simulink model "MOBATSim"  (R2020b)
settings: Solver=FixedStepAuto  StartTime=0.0  StopTime=Sim_t  FixedStep=0.01  MinStep=0.01  RelTol=1e-2
values from neighbouring files (symbols this model uses):
  Vehicles = evalin('base','Vehicles')    [I2V.m]    (also in VehicleSensors.m)
undefined symbols (not defined in the file or in its folder): Sim_Ts
libraries: simulink x50, robotalgslib x10, drivingvehiclecontroller x10, mpcadaslib x10, pid_lib x10
(part 2 of 7)

== system MOBATSim/Vehicle Model 9 ==
  note: Perception
  note: Decision-Making
  note: Control
  Behavioural Planner : MATLABSystem  System=VehicleDrivingMode  Vehicle_id=Vehicle_id  SimulateUsing=Interpreted execution
      mask Type: VehicleDrivingMode
      mask Display:
      | image('MOBATSIM-Icon-Set_7- Behavioural Planner.png');
      | port_label('input',1,'vehicleDetected');
      | port_label('output',1,'SpeedReference');
      | port_label('output',2,'DistanceReference');
      | port_label('output',3,'LeadSpeed');
      | port_label('output',4,'DrivingMode');
      | port_label('output',5,'Dist2Stop');
      | port_label('output',6,'laneChange');
  Longitudinal and Lateral Controllers : Subsystem
  Path Planner : Subsystem  Variant=on  VariantControlMode=label  LabelModeActiveChoice=Astar  mask{PathPlanningAlgorithm=Astar}
      mask prompts: PathPlanningAlgorithm "Path Planning Algorithm"
      mask TypeOptions PathPlanningAlgorithm: Astar | ShortestPathFinder
      mask Callback PathPlanningAlgorithm: set_param(gcb,'OverrideUsingVariant',get_param(gcb,'PathPlanningAlgorithm'));
      mask Display: image("MOBATSIM-Icon-Set_8- Navigation.png");
  Transform to MOBATSim Coordinates : Subsystem
  Vehicle Model : Subsystem  mask{Vehicle_id=Vehicle_id}
      mask prompts: Vehicle_id "Vehicle ID"
      mask Display: image('MOBATSIM-Icon-Set_13- VehicleModel.png'); % Use "Edit Image" on toolstrip to change.
  Vehicle Sensors : MATLABSystem  System=VehicleSensors  Vehicle_id=Vehicle_id  Tsample=Sim_Ts  OffsetTime=0  SimulateUsing=Interpreted execution
      mask Type: VehicleSensors
      mask Display:
      | image('MOBATSIM-Icon-Set_4- Sensor.png');
      | port_label('output',1,'V2VcommIDs');
      | port_label('output',2,'vehicleDetected');
  Vehicle Status Check and Acceleration to Speed : Subsystem
  Vehicle V2I Output : MATLABSystem  System=VehicleV2I_Out  Vehicle_id=Vehicle_id  SimulateUsing=Interpreted execution
      mask Type: VehicleV2I_Out
      mask Display:
      | image('MOBATSIM-Icon-Set_6- V2l.png');
      | port_label('input',1,'waypointReached');
      | port_label('output',1,'V2Idata');
  Position : Outport  VectorParamsAs1DForOutWhenUnconnected=off
  Orientation : Outport  Port=2  VectorParamsAs1DForOutWhenUnconnected=off
  Speed : Outport  Port=3  VectorParamsAs1DForOutWhenUnconnected=off
  V_Network_Out : Outport  Port=4  VectorParamsAs1DForOutWhenUnconnected=off
  wires:
  Vehicle V2I Output/1 -> V_Network_Out/1
  Vehicle Sensors/2 -> Behavioural Planner/1
  Behavioural Planner/1 -> Longitudinal and Lateral Controllers/1(Speed Reference)
  Behavioural Planner/2 -> Longitudinal and Lateral Controllers/2(Inter Vehicular Distance)
  Behavioural Planner/3 -> Longitudinal and Lateral Controllers/3(Lead Speed)
  Behavioural Planner/4 -> Longitudinal and Lateral Controllers/4(drivingMode)
  Behavioural Planner/5 -> Longitudinal and Lateral Controllers/5(Dist2Stop)
  Transform to MOBATSim Coordinates/1(Position) -> Position/1
  Transform to MOBATSim Coordinates/2(Orientation) -> Orientation/1
  Vehicle Model/2(Speed) -> Longitudinal and Lateral Controllers/8(Actual Speed), Speed/1
  Vehicle Model/1(Pose) -> Longitudinal and Lateral Controllers/7(Actual Pose), Transform to MOBATSim Coordinates/1(Pose)
  Longitudinal and Lateral Controllers/1(Longitudinal Acceleration Cmd) -> Vehicle Status Check and Acceleration to Speed/1(Reference Acceleration)
  Longitudinal and Lateral Controllers/2(Reference Steering Angle) -> Vehicle Status Check and Acceleration to Speed/2(Reference Steering Angle)
  Vehicle Status Check and Acceleration to Speed/2(Steering Angle Cmd) -> Vehicle Model/2(Steering Angle)
  Behavioural Planner/6 -> Longitudinal and Lateral Controllers/6(laneChange)
  Vehicle Sensors/1 -> Path Planner/1(CommunicationIDs)
  Path Planner/1(waypointReached) -> Vehicle V2I Output/1
  Vehicle Status Check and Acceleration to Speed/1(Speed Cmd) -> Vehicle Model/1(Longitudinal Speed)

== system MOBATSim/Vehicle Model 1/Longitudinal and Lateral Controllers ==
  Speed Reference : Inport
  Inter Vehicular Distance : Inport  Port=2
  Lead Speed : Inport  Port=3
  drivingMode : Inport  Port=4
  Dist2Stop : Inport  Port=5
  laneChange : Inport  Port=6
  Actual Pose : Inport  Port=7
  Actual Speed : Inport  Port=8
  Lateral Motion Control : Subsystem  Variant=on  VariantControlMode=label  LabelModeActiveChoice=STANLEY  mask{modeLateral=STANLEY}
      mask prompts: modeLateral "Lateral Control Mode:"
      mask TypeOptions modeLateral: PURE_PURSUIT | STANLEY
      mask Callback modeLateral: set_param(gcb,'OverrideUsingVariant',get_param(gcb,'modeLateral'));
  Longitudinal Speed Control : Subsystem
  Longitudinal Acceleration Cmd : Outport
  Reference Steering Angle : Outport  Port=2
  wires:
  laneChange/1 -> Lateral Motion Control/3(changeLane)
  Lateral Motion Control/1(SteerCmd) -> Reference Steering Angle/1
  Actual Speed/1 -> Lateral Motion Control/1(speed), Longitudinal Speed Control/6(Actual Speed)
  drivingMode/1 -> Longitudinal Speed Control/4(Driving Mode)
  Longitudinal Speed Control/1(Longitduinal Acceleration Command) -> Longitudinal Acceleration Cmd/1
  Dist2Stop/1 -> Longitudinal Speed Control/5(Dist2Stop)
  Inter Vehicular Distance/1 -> Longitudinal Speed Control/2(Inter Vehicular Distance)
  Lead Speed/1 -> Longitudinal Speed Control/3(Lead Speed)
  Speed Reference/1 -> Longitudinal Speed Control/1(Speed Reference)
  Actual Pose/1 -> Lateral Motion Control/2(pose)

== system MOBATSim/Vehicle Model 1/Path Planner ==
  note: 1) Add Subsystem or Model blocks as valid variant choices.
      | 2) You cannot connect blocks at this level. At simulation, connectivity is automatically
      | determined, based on the active variant and port name matching.
  CommunicationIDs : Inport
  Astar : Subsystem  VariantControl=Astar
  ShortestPathFinder : Subsystem  VariantControl=ShortestPathFinder
  waypointReached : Outport

== system MOBATSim/Vehicle Model 1/Transform to MOBATSim Coordinates ==
  Pose : Inport
  Constant : Constant  Value=0
  Constant1 : Constant
  Constant2 : Constant  Value=0
  Constant3 : Constant  Value=0
  Constant4 : Constant  Value=pi/2
  Gain : Gain  Gain=-1
  Matrix Concatenate : Concatenate  NumInputs=4  ConcatenateDimension=2
  Matrix Concatenate1 : Concatenate  NumInputs=3  ConcatenateDimension=2
  Selector1 : Selector  InputPortWidth=3  IndexOptions=Index vector (dialog)  Indices=[3]  OutputSizes=1
  Selector3 : Selector  InputPortWidth=3  IndexOptions=Index vector (dialog)  Indices=[1]  OutputSizes=1
  Selector4 : Selector  InputPortWidth=3  IndexOptions=Index vector (dialog)  Indices=[2]  OutputSizes=1
  Sum : Sum  Inputs=|++
  Position : Outport
  Orientation : Outport  Port=2
  wires:
  Sum/1 -> Matrix Concatenate/4
  Constant2/1 -> Matrix Concatenate/1
  Constant3/1 -> Matrix Concatenate1/2
  Gain/1 -> Matrix Concatenate1/3
  Constant4/1 -> Sum/2
  Constant1/1 -> Matrix Concatenate/2
  Selector1/1 -> Sum/1
  Constant/1 -> Matrix Concatenate/3
  Matrix Concatenate/1 -> Orientation/1
  Matrix Concatenate1/1 -> Position/1
  Selector4/1 -> Gain/1
  Selector3/1 -> Matrix Concatenate1/1
  Pose/1 -> Selector1/1, Selector4/1, Selector3/1

== system MOBATSim/Vehicle Model 1/Vehicle Model ==
  Longitudinal Speed : Inport
  Steering Angle : Inport  Port=2
  Delay : Delay  DelayLength=1  SampleTime=Sim_Ts
  Kinematic Bicycle Model : Subsystem
  Selector3 : Selector  InputPortWidth=3  IndexOptions=Index vector (dialog)  Indices=[1]  OutputSizes=1
  Selector4 : Selector  InputPortWidth=3  IndexOptions=Index vector (dialog)  Indices=[2]  OutputSizes=1
  Sqrt : Sqrt  SaturateOnIntegerOverflow=on
  Square : Math  Operator=square  SaturateOnIntegerOverflow=on
  Square1 : Math  Operator=square  SaturateOnIntegerOverflow=on
  Sum1 : Sum  Inputs=|++
  Zero-Order Hold1 : ZeroOrderHold  SampleTime=Sim_Ts
  Zero-Order Hold2 : ZeroOrderHold  SampleTime=Sim_Ts
  Pose : Outport
  Speed : Outport  Port=2
  wires:
  Delay/1 -> Speed/1
  Kinematic Bicycle Model/1(state) -> Zero-Order Hold1/1
  Selector4/1 -> Square1/1
  Longitudinal Speed/1 -> Kinematic Bicycle Model/1(v)
  Steering Angle/1 -> Kinematic Bicycle Model/2(Steering Angle)
  Sum1/1 -> Sqrt/1
  Sqrt/1 -> Delay/1
  Square/1 -> Sum1/1
  Square1/1 -> Sum1/2
  Selector3/1 -> Square/1
  Kinematic Bicycle Model/2(stateDot) -> Zero-Order Hold2/1
  Zero-Order Hold1/1 -> Pose/1
  Zero-Order Hold2/1 -> Selector4/1, Selector3/1

== system MOBATSim/Vehicle Model 1/Vehicle Status Check and Acceleration to Speed ==
  note: Longitudinal
  Reference Acceleration : Inport
  Reference Steering Angle : Inport  Port=2
  Acceleration to Speed : Integrator  LimitOutput=on  LowerSaturationLimit=0
  MATLAB System : MATLABSystem  System=VehicleStopStatusCheck  Vehicle_id=Vehicle_id  SimulateUsing=Interpreted execution
      mask Type: VehicleStopStatusCheck
      mask Display:
      | disp('VehicleStopStatusCheck');
      | port_label('input',1,'Acc');
      | port_label('input',2,'Steering');
      | port_label('output',1,'Acc');
      | port_label('output',2,'Stop');
      | port_label('output',3,'Steering');
  Product : Product
  Signal Specification : SignalSpecification  Dimensions=1
  Stop Check : simulink/Logic and Bit Operations/Compare To Constant  relop=~=  const=1  OutDataTypeStr=uint8
  Zero-Order Hold : ZeroOrderHold  SampleTime=Sim_Ts
  Speed Cmd : Outport
  Steering Angle Cmd : Outport  Port=2
  wires:
  Acceleration to Speed/1 -> Signal Specification/1
  Stop Check/1 -> Product/2
  MATLAB System/3 -> Steering Angle Cmd/1
  Signal Specification/1 -> Zero-Order Hold/1
  Reference Acceleration/1 -> MATLAB System/1
  Zero-Order Hold/1 -> Product/1
  Product/1 -> Speed Cmd/1
  MATLAB System/1 -> Acceleration to Speed/1
  Reference Steering Angle/1 -> MATLAB System/2
  MATLAB System/2 -> Stop Check/1

== system MOBATSim/Vehicle Model 10/Longitudinal and Lateral Controllers ==
  Speed Reference : Inport
  Inter Vehicular Distance : Inport  Port=2
  Lead Speed : Inport  Port=3
  drivingMode : Inport  Port=4
  Dist2Stop : Inport  Port=5
  laneChange : Inport  Port=6
  Actual Pose : Inport  Port=7
  Actual Speed : Inport  Port=8
  Lateral Motion Control : Subsystem  Variant=on  VariantControlMode=label  LabelModeActiveChoice=STANLEY  mask{modeLateral=STANLEY}
      mask prompts: modeLateral "Lateral Control Mode:"
      mask TypeOptions modeLateral: PURE_PURSUIT | STANLEY
      mask Callback modeLateral: set_param(gcb,'OverrideUsingVariant',get_param(gcb,'modeLateral'));
  Longitudinal Speed Control : Subsystem
  Longitudinal Acceleration Cmd : Outport
  Reference Steering Angle : Outport  Port=2
  wires:
  laneChange/1 -> Lateral Motion Control/3(changeLane)
  Lateral Motion Control/1(SteerCmd) -> Reference Steering Angle/1
  Actual Speed/1 -> Lateral Motion Control/1(speed), Longitudinal Speed Control/6(Actual Speed)
  drivingMode/1 -> Longitudinal Speed Control/4(Driving Mode)
  Longitudinal Speed Control/1(Longitduinal Acceleration Command) -> Longitudinal Acceleration Cmd/1
  Dist2Stop/1 -> Longitudinal Speed Control/5(Dist2Stop)
  Inter Vehicular Distance/1 -> Longitudinal Speed Control/2(Inter Vehicular Distance)
  Lead Speed/1 -> Longitudinal Speed Control/3(Lead Speed)
  Speed Reference/1 -> Longitudinal Speed Control/1(Speed Reference)
  Actual Pose/1 -> Lateral Motion Control/2(pose)

== system MOBATSim/Vehicle Model 10/Path Planner ==
  note: 1) Add Subsystem or Model blocks as valid variant choices.
      | 2) You cannot connect blocks at this level. At simulation, connectivity is automatically
      | determined, based on the active variant and port name matching.
  CommunicationIDs : Inport
  Astar : Subsystem  VariantControl=Astar
  ShortestPathFinder : Subsystem  VariantControl=ShortestPathFinder
  waypointReached : Outport

== system MOBATSim/Vehicle Model 10/Transform to MOBATSim Coordinates ==
  Pose : Inport
  Constant : Constant  Value=0
  Constant1 : Constant
  Constant2 : Constant  Value=0
  Constant3 : Constant  Value=0
  Constant4 : Constant  Value=pi/2
  Gain : Gain  Gain=-1
  Matrix Concatenate : Concatenate  NumInputs=4  ConcatenateDimension=2
  Matrix Concatenate1 : Concatenate  NumInputs=3  ConcatenateDimension=2
  Selector1 : Selector  InputPortWidth=3  IndexOptions=Index vector (dialog)  Indices=[3]  OutputSizes=1
  Selector3 : Selector  InputPortWidth=3  IndexOptions=Index vector (dialog)  Indices=[1]  OutputSizes=1
  Selector4 : Selector  InputPortWidth=3  IndexOptions=Index vector (dialog)  Indices=[2]  OutputSizes=1
  Sum : Sum  Inputs=|++
  Position : Outport
  Orientation : Outport  Port=2
  wires:
  Sum/1 -> Matrix Concatenate/4
  Constant2/1 -> Matrix Concatenate/1
  Constant3/1 -> Matrix Concatenate1/2
  Gain/1 -> Matrix Concatenate1/3
  Constant4/1 -> Sum/2
  Constant1/1 -> Matrix Concatenate/2
  Selector1/1 -> Sum/1
  Constant/1 -> Matrix Concatenate/3
  Matrix Concatenate/1 -> Orientation/1
  Matrix Concatenate1/1 -> Position/1
  Selector4/1 -> Gain/1
  Selector3/1 -> Matrix Concatenate1/1
  Pose/1 -> Selector1/1, Selector4/1, Selector3/1

== system MOBATSim/Vehicle Model 10/Vehicle Model ==
  Longitudinal Speed : Inport
  Steering Angle : Inport  Port=2
  Delay : Delay  DelayLength=1  SampleTime=Sim_Ts
  Kinematic Bicycle Model : Subsystem
  Selector3 : Selector  InputPortWidth=3  IndexOptions=Index vector (dialog)  Indices=[1]  OutputSizes=1
  Selector4 : Selector  InputPortWidth=3  IndexOptions=Index vector (dialog)  Indices=[2]  OutputSizes=1
  Sqrt : Sqrt  SaturateOnIntegerOverflow=on
  Square : Math  Operator=square  SaturateOnIntegerOverflow=on
  Square1 : Math  Operator=square  SaturateOnIntegerOverflow=on
  Sum1 : Sum  Inputs=|++
  Zero-Order Hold1 : ZeroOrderHold  SampleTime=Sim_Ts
  Zero-Order Hold2 : ZeroOrderHold  SampleTime=Sim_Ts
  Pose : Outport
  Speed : Outport  Port=2
  wires:
  Delay/1 -> Speed/1
  Kinematic Bicycle Model/1(state) -> Zero-Order Hold1/1
  Selector4/1 -> Square1/1
  Longitudinal Speed/1 -> Kinematic Bicycle Model/1(v)
  Steering Angle/1 -> Kinematic Bicycle Model/2(Steering Angle)
  Sum1/1 -> Sqrt/1
  Sqrt/1 -> Delay/1
  Square/1 -> Sum1/1
  Square1/1 -> Sum1/2
  Selector3/1 -> Square/1
  Kinematic Bicycle Model/2(stateDot) -> Zero-Order Hold2/1
  Zero-Order Hold1/1 -> Pose/1
  Zero-Order Hold2/1 -> Selector4/1, Selector3/1

== system MOBATSim/Vehicle Model 10/Vehicle Status Check and Acceleration to Speed ==
  note: Longitudinal
  Reference Acceleration : Inport
  Reference Steering Angle : Inport  Port=2
  Acceleration to Speed : Integrator  LimitOutput=on  LowerSaturationLimit=0
  MATLAB System : MATLABSystem  System=VehicleStopStatusCheck  Vehicle_id=Vehicle_id  SimulateUsing=Interpreted execution
      mask Type: VehicleStopStatusCheck
      mask Display:
      | disp('VehicleStopStatusCheck');
      | port_label('input',1,'Acc');
      | port_label('input',2,'Steering');
      | port_label('output',1,'Acc');
      | port_label('output',2,'Stop');
      | port_label('output',3,'Steering');
  Product : Product
  Signal Specification : SignalSpecification  Dimensions=1
  Stop Check : simulink/Logic and Bit Operations/Compare To Constant  relop=~=  const=1  OutDataTypeStr=uint8
  Zero-Order Hold : ZeroOrderHold  SampleTime=Sim_Ts
  Speed Cmd : Outport
  Steering Angle Cmd : Outport  Port=2
  wires:
  Acceleration to Speed/1 -> Signal Specification/1
  Stop Check/1 -> Product/2
  MATLAB System/3 -> Steering Angle Cmd/1
  Signal Specification/1 -> Zero-Order Hold/1
  Reference Acceleration/1 -> MATLAB System/1
  Zero-Order Hold/1 -> Product/1
  Product/1 -> Speed Cmd/1
  MATLAB System/1 -> Acceleration to Speed/1
  Reference Steering Angle/1 -> MATLAB System/2
  MATLAB System/2 -> Stop Check/1

== system MOBATSim/Vehicle Model 2/Longitudinal and Lateral Controllers ==
  Speed Reference : Inport
  Inter Vehicular Distance : Inport  Port=2
  Lead Speed : Inport  Port=3
  Driving Mode : Inport  Port=4
  Dist2Stop : Inport  Port=5
  laneChange : Inport  Port=6
  Actual Pose : Inport  Port=7
  Actual Speed : Inport  Port=8
  Lateral Motion Control : Subsystem  Variant=on  VariantControlMode=label  LabelModeActiveChoice=STANLEY  mask{modeLateral=STANLEY}
      mask prompts: modeLateral "Lateral Control Mode:"
      mask TypeOptions modeLateral: PURE_PURSUIT | STANLEY
      mask Callback modeLateral: set_param(gcb,'OverrideUsingVariant',get_param(gcb,'modeLateral'));
  Longitudinal Speed Control : Subsystem
  Longitudinal Acceleration Cmd : Outport
  Reference Steering Angle : Outport  Port=2
  wires:
  Driving Mode/1 -> Longitudinal Speed Control/4(Driving Mode)
  Inter Vehicular Distance/1 -> Longitudinal Speed Control/2(Inter Vehicular Distance)
  Speed Reference/1 -> Longitudinal Speed Control/1(Speed Reference)
  Lead Speed/1 -> Longitudinal Speed Control/3(Lead Speed)
  Dist2Stop/1 -> Longitudinal Speed Control/5(Dist2Stop)
  Actual Speed/1 -> Lateral Motion Control/1(speed), Longitudinal Speed Control/6(Actual Speed)
  Longitudinal Speed Control/1(Longitduinal Acceleration Command) -> Longitudinal Acceleration Cmd/1
  laneChange/1 -> Lateral Motion Control/3(changeLane)
  Actual Pose/1 -> Lateral Motion Control/2(pose)
  Lateral Motion Control/1(SteerCmd) -> Reference Steering Angle/1

== system MOBATSim/Vehicle Model 2/Path Planner ==
  note: 1) Add Subsystem or Model blocks as valid variant choices.
      | 2) You cannot connect blocks at this level. At simulation, connectivity is automatically
      | determined, based on the active variant and port name matching.
  CommunicationIDs : Inport
  Astar : Subsystem  VariantControl=Astar
  ShortestPathFinder : Subsystem  VariantControl=ShortestPathFinder
  waypointReached : Outport

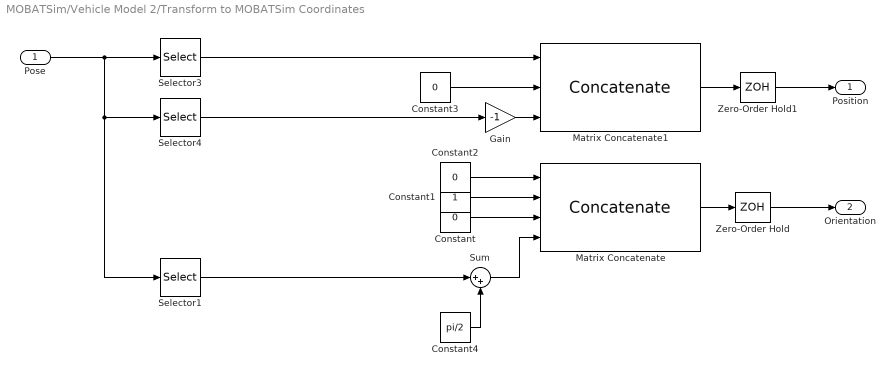
== system MOBATSim/Vehicle Model 2/Transform to MOBATSim Coordinates ==
  Pose : Inport
  Constant : Constant  Value=0
  Constant1 : Constant
  Constant2 : Constant  Value=0
  Constant3 : Constant  Value=0
  Constant4 : Constant  Value=pi/2
  Gain : Gain  Gain=-1
  Matrix Concatenate : Concatenate  NumInputs=4  ConcatenateDimension=2
  Matrix Concatenate1 : Concatenate  NumInputs=3  ConcatenateDimension=2
  Selector1 : Selector  InputPortWidth=3  IndexOptions=Index vector (dialog)  Indices=[3]  OutputSizes=1
  Selector3 : Selector  InputPortWidth=3  IndexOptions=Index vector (dialog)  Indices=[1]  OutputSizes=1
  Selector4 : Selector  InputPortWidth=3  IndexOptions=Index vector (dialog)  Indices=[2]  OutputSizes=1
  Sum : Sum  Inputs=|++
  Zero-Order Hold : ZeroOrderHold  SampleTime=Sim_Ts
  Zero-Order Hold1 : ZeroOrderHold  SampleTime=Sim_Ts
  Position : Outport
  Orientation : Outport  Port=2
  wires:
  Sum/1 -> Matrix Concatenate/4
  Constant2/1 -> Matrix Concatenate/1
  Matrix Concatenate/1 -> Zero-Order Hold/1
  Constant3/1 -> Matrix Concatenate1/2
  Gain/1 -> Matrix Concatenate1/3
  Constant4/1 -> Sum/2
  Constant1/1 -> Matrix Concatenate/2
  Matrix Concatenate1/1 -> Zero-Order Hold1/1
  Selector1/1 -> Sum/1
  Constant/1 -> Matrix Concatenate/3
  Zero-Order Hold/1 -> Orientation/1
  Zero-Order Hold1/1 -> Position/1
  Selector4/1 -> Gain/1
  Selector3/1 -> Matrix Concatenate1/1
  Pose/1 -> Selector1/1, Selector4/1, Selector3/1

== system MOBATSim/Vehicle Model 2/Vehicle Model ==
  Longitudinal Speed : Inport
  Steering Angle : Inport  Port=2
  Delay : Delay  DelayLength=1  SampleTime=Sim_Ts
  Kinematic Bicycle Model : Subsystem
  Selector3 : Selector  InputPortWidth=3  IndexOptions=Index vector (dialog)  Indices=[1]  OutputSizes=1
  Selector4 : Selector  InputPortWidth=3  IndexOptions=Index vector (dialog)  Indices=[2]  OutputSizes=1
  Sqrt : Sqrt  SaturateOnIntegerOverflow=on
  Square : Math  Operator=square  SaturateOnIntegerOverflow=on
  Square1 : Math  Operator=square  SaturateOnIntegerOverflow=on
  Sum1 : Sum  Inputs=|++
  Zero-Order Hold1 : ZeroOrderHold  SampleTime=Sim_Ts
  Zero-Order Hold2 : ZeroOrderHold  SampleTime=Sim_Ts
  Pose : Outport
  Speed : Outport  Port=2
  wires:
  Delay/1 -> Speed/1
  Kinematic Bicycle Model/1(state) -> Zero-Order Hold1/1
  Selector4/1 -> Square1/1
  Longitudinal Speed/1 -> Kinematic Bicycle Model/1(v)
  Steering Angle/1 -> Kinematic Bicycle Model/2(Steering Angle)
  Sum1/1 -> Sqrt/1
  Sqrt/1 -> Delay/1
  Square/1 -> Sum1/1
  Square1/1 -> Sum1/2
  Selector3/1 -> Square/1
  Kinematic Bicycle Model/2(stateDot) -> Zero-Order Hold2/1
  Zero-Order Hold1/1 -> Pose/1
  Zero-Order Hold2/1 -> Selector4/1, Selector3/1

== system MOBATSim/Vehicle Model 2/Vehicle Status Check and Acceleration to Speed ==
  note: Longitudinal
  Reference Acceleration : Inport
  Reference Steering Angle : Inport  Port=2
  Acceleration to Speed : Integrator  LimitOutput=on  UpperSaturationLimit=Vehicles(Vehicle_id).dynamics.maxSpeed  LowerSaturationLimit=0
  MATLAB System : MATLABSystem  System=VehicleStopStatusCheck  Vehicle_id=Vehicle_id  SimulateUsing=Interpreted execution
      mask Type: VehicleStopStatusCheck
      mask Display:
      | disp('VehicleStopStatusCheck');
      | port_label('input',1,'Acc');
      | port_label('input',2,'Steering');
      | port_label('output',1,'Acc');
      | port_label('output',2,'Stop');
      | port_label('output',3,'Steering');
  Product : Product
  Signal Specification : SignalSpecification  Dimensions=1
  Stop Check : simulink/Logic and Bit Operations/Compare To Constant  relop=~=  const=1  OutDataTypeStr=uint8
  Zero-Order Hold : ZeroOrderHold  SampleTime=Sim_Ts
  Speed Cmd : Outport
  Steering Angle Cmd : Outport  Port=2
  wires:
  Acceleration to Speed/1 -> Signal Specification/1
  Stop Check/1 -> Product/2
  Signal Specification/1 -> Zero-Order Hold/1
  Reference Acceleration/1 -> MATLAB System/1
  Zero-Order Hold/1 -> Product/1
  Product/1 -> Speed Cmd/1
  MATLAB System/1 -> Acceleration to Speed/1
  Reference Steering Angle/1 -> MATLAB System/2
  MATLAB System/3 -> Steering Angle Cmd/1
  MATLAB System/2 -> Stop Check/1

== system MOBATSim/Vehicle Model 3/Longitudinal and Lateral Controllers ==
  Speed Reference : Inport
  Inter Vehicular Distance : Inport  Port=2
  Lead Speed : Inport  Port=3
  drivingMode : Inport  Port=4
  Dist2Stop : Inport  Port=5
  laneChange : Inport  Port=6
  Actual Pose : Inport  Port=7
  Actual Speed : Inport  Port=8
  Lateral Motion Control : Subsystem  Variant=on  VariantControlMode=label  LabelModeActiveChoice=STANLEY  mask{modeLateral=STANLEY}
      mask prompts: modeLateral "Lateral Control Mode:"
      mask TypeOptions modeLateral: PURE_PURSUIT | STANLEY
      mask Callback modeLateral: set_param(gcb,'OverrideUsingVariant',get_param(gcb,'modeLateral'));
  Longitudinal Speed Control : Subsystem
  Longitudinal Acceleration Cmd : Outport
  Reference Steering Angle : Outport  Port=2
  wires:
  laneChange/1 -> Lateral Motion Control/3(changeLane)
  Lateral Motion Control/1(SteerCmd) -> Reference Steering Angle/1
  Actual Speed/1 -> Lateral Motion Control/1(speed), Longitudinal Speed Control/6(Actual Speed)
  drivingMode/1 -> Longitudinal Speed Control/4(Driving Mode)
  Longitudinal Speed Control/1(Longitduinal Acceleration Command) -> Longitudinal Acceleration Cmd/1
  Dist2Stop/1 -> Longitudinal Speed Control/5(Dist2Stop)
  Inter Vehicular Distance/1 -> Longitudinal Speed Control/2(Inter Vehicular Distance)
  Lead Speed/1 -> Longitudinal Speed Control/3(Lead Speed)
  Speed Reference/1 -> Longitudinal Speed Control/1(Speed Reference)
  Actual Pose/1 -> Lateral Motion Control/2(pose)

== system MOBATSim/Vehicle Model 3/Path Planner ==
  note: 1) Add Subsystem or Model blocks as valid variant choices.
      | 2) You cannot connect blocks at this level. At simulation, connectivity is automatically
      | determined, based on the active variant and port name matching.
  CommunicationIDs : Inport
  Astar : Subsystem  VariantControl=Astar
  ShortestPathFinder : Subsystem  VariantControl=ShortestPathFinder
  waypointReached : Outport

== system MOBATSim/Vehicle Model 3/Transform to MOBATSim Coordinates ==
  Pose : Inport
  Constant : Constant  Value=0
  Constant1 : Constant
  Constant2 : Constant  Value=0
  Constant3 : Constant  Value=0
  Constant4 : Constant  Value=pi/2
  Gain : Gain  Gain=-1
  Matrix Concatenate : Concatenate  NumInputs=4  ConcatenateDimension=2
  Matrix Concatenate1 : Concatenate  NumInputs=3  ConcatenateDimension=2
  Selector1 : Selector  InputPortWidth=3  IndexOptions=Index vector (dialog)  Indices=[3]  OutputSizes=1
  Selector3 : Selector  InputPortWidth=3  IndexOptions=Index vector (dialog)  Indices=[1]  OutputSizes=1
  Selector4 : Selector  InputPortWidth=3  IndexOptions=Index vector (dialog)  Indices=[2]  OutputSizes=1
  Sum : Sum  Inputs=|++
  Position : Outport
  Orientation : Outport  Port=2
  wires:
  Sum/1 -> Matrix Concatenate/4
  Constant2/1 -> Matrix Concatenate/1
  Constant3/1 -> Matrix Concatenate1/2
  Gain/1 -> Matrix Concatenate1/3
  Constant4/1 -> Sum/2
  Constant1/1 -> Matrix Concatenate/2
  Selector1/1 -> Sum/1
  Constant/1 -> Matrix Concatenate/3
  Matrix Concatenate/1 -> Orientation/1
  Matrix Concatenate1/1 -> Position/1
  Selector4/1 -> Gain/1
  Selector3/1 -> Matrix Concatenate1/1
  Pose/1 -> Selector1/1, Selector4/1, Selector3/1

== system MOBATSim/Vehicle Model 3/Vehicle Model ==
  Longitudinal Speed : Inport
  Steering Angle : Inport  Port=2
  Delay : Delay  DelayLength=1  SampleTime=Sim_Ts
  Kinematic Bicycle Model : Subsystem
  Selector3 : Selector  InputPortWidth=3  IndexOptions=Index vector (dialog)  Indices=[1]  OutputSizes=1
  Selector4 : Selector  InputPortWidth=3  IndexOptions=Index vector (dialog)  Indices=[2]  OutputSizes=1
  Sqrt : Sqrt  SaturateOnIntegerOverflow=on
  Square : Math  Operator=square  SaturateOnIntegerOverflow=on
  Square1 : Math  Operator=square  SaturateOnIntegerOverflow=on
  Sum1 : Sum  Inputs=|++
  Zero-Order Hold1 : ZeroOrderHold  SampleTime=Sim_Ts
  Zero-Order Hold2 : ZeroOrderHold  SampleTime=Sim_Ts
  Pose : Outport
  Speed : Outport  Port=2
  wires:
  Delay/1 -> Speed/1
  Kinematic Bicycle Model/1(state) -> Zero-Order Hold1/1
  Selector4/1 -> Square1/1
  Longitudinal Speed/1 -> Kinematic Bicycle Model/1(v)
  Steering Angle/1 -> Kinematic Bicycle Model/2(Steering Angle)
  Sum1/1 -> Sqrt/1
  Sqrt/1 -> Delay/1
  Square/1 -> Sum1/1
  Square1/1 -> Sum1/2
  Selector3/1 -> Square/1
  Kinematic Bicycle Model/2(stateDot) -> Zero-Order Hold2/1
  Zero-Order Hold1/1 -> Pose/1
  Zero-Order Hold2/1 -> Selector4/1, Selector3/1

== system MOBATSim/Vehicle Model 3/Vehicle Status Check and Acceleration to Speed ==
  note: Longitudinal
  Reference Acceleration : Inport
  Reference Steering Angle : Inport  Port=2
  Acceleration to Speed : Integrator  LimitOutput=on  LowerSaturationLimit=0
  MATLAB System : MATLABSystem  System=VehicleStopStatusCheck  Vehicle_id=Vehicle_id  SimulateUsing=Interpreted execution
      mask Type: VehicleStopStatusCheck
      mask Display:
      | disp('VehicleStopStatusCheck');
      | port_label('input',1,'Acc');
      | port_label('input',2,'Steering');
      | port_label('output',1,'Acc');
      | port_label('output',2,'Stop');
      | port_label('output',3,'Steering');
  Product : Product
  Signal Specification : SignalSpecification  Dimensions=1
  Stop Check : simulink/Logic and Bit Operations/Compare To Constant  relop=~=  const=1  OutDataTypeStr=uint8
  Zero-Order Hold : ZeroOrderHold  SampleTime=Sim_Ts
  Speed Cmd : Outport
  Steering Angle Cmd : Outport  Port=2
  wires:
  Acceleration to Speed/1 -> Signal Specification/1
  Stop Check/1 -> Product/2
  MATLAB System/3 -> Steering Angle Cmd/1
  Signal Specification/1 -> Zero-Order Hold/1
  Reference Acceleration/1 -> MATLAB System/1
  Zero-Order Hold/1 -> Product/1
  Product/1 -> Speed Cmd/1
  MATLAB System/1 -> Acceleration to Speed/1
  Reference Steering Angle/1 -> MATLAB System/2
  MATLAB System/2 -> Stop Check/1

== system MOBATSim/Vehicle Model 4/Longitudinal and Lateral Controllers ==
  Speed Reference : Inport
  Inter Vehicular Distance : Inport  Port=2
  Lead Speed : Inport  Port=3
  drivingMode : Inport  Port=4
  Dist2Stop : Inport  Port=5
  laneChange : Inport  Port=6
  Actual Pose : Inport  Port=7
  Actual Speed : Inport  Port=8
  Lateral Motion Control : Subsystem  Variant=on  VariantControlMode=label  LabelModeActiveChoice=STANLEY  mask{modeLateral=STANLEY}
      mask prompts: modeLateral "Lateral Control Mode:"
      mask TypeOptions modeLateral: PURE_PURSUIT | STANLEY
      mask Callback modeLateral: set_param(gcb,'OverrideUsingVariant',get_param(gcb,'modeLateral'));
  Longitudinal Speed Control : Subsystem
  Longitudinal Acceleration Cmd : Outport
  Reference Steering Angle : Outport  Port=2
  wires:
  laneChange/1 -> Lateral Motion Control/3(changeLane)
  Lateral Motion Control/1(SteerCmd) -> Reference Steering Angle/1
  Actual Speed/1 -> Lateral Motion Control/1(speed), Longitudinal Speed Control/6(Actual Speed)
  drivingMode/1 -> Longitudinal Speed Control/4(Driving Mode)
  Longitudinal Speed Control/1(Longitduinal Acceleration Command) -> Longitudinal Acceleration Cmd/1
  Dist2Stop/1 -> Longitudinal Speed Control/5(Dist2Stop)
  Inter Vehicular Distance/1 -> Longitudinal Speed Control/2(Inter Vehicular Distance)
  Lead Speed/1 -> Longitudinal Speed Control/3(Lead Speed)
  Speed Reference/1 -> Longitudinal Speed Control/1(Speed Reference)
  Actual Pose/1 -> Lateral Motion Control/2(pose)

== system MOBATSim/Vehicle Model 4/Path Planner ==
  note: 1) Add Subsystem or Model blocks as valid variant choices.
      | 2) You cannot connect blocks at this level. At simulation, connectivity is automatically
      | determined, based on the active variant and port name matching.
  CommunicationIDs : Inport
  Astar : Subsystem  VariantControl=Astar
  ShortestPathFinder : Subsystem  VariantControl=ShortestPathFinder
  waypointReached : Outport

== system MOBATSim/Vehicle Model 4/Transform to MOBATSim Coordinates ==
  Pose : Inport
  Constant : Constant  Value=0
  Constant1 : Constant
  Constant2 : Constant  Value=0
  Constant3 : Constant  Value=0
  Constant4 : Constant  Value=pi/2
  Gain : Gain  Gain=-1
  Matrix Concatenate : Concatenate  NumInputs=4  ConcatenateDimension=2
  Matrix Concatenate1 : Concatenate  NumInputs=3  ConcatenateDimension=2
  Selector1 : Selector  InputPortWidth=3  IndexOptions=Index vector (dialog)  Indices=[3]  OutputSizes=1
  Selector3 : Selector  InputPortWidth=3  IndexOptions=Index vector (dialog)  Indices=[1]  OutputSizes=1
  Selector4 : Selector  InputPortWidth=3  IndexOptions=Index vector (dialog)  Indices=[2]  OutputSizes=1
  Sum : Sum  Inputs=|++
  Position : Outport
  Orientation : Outport  Port=2
  wires:
  Sum/1 -> Matrix Concatenate/4
  Constant2/1 -> Matrix Concatenate/1
  Constant3/1 -> Matrix Concatenate1/2
  Gain/1 -> Matrix Concatenate1/3
  Constant4/1 -> Sum/2
  Constant1/1 -> Matrix Concatenate/2
  Selector1/1 -> Sum/1
  Constant/1 -> Matrix Concatenate/3
  Matrix Concatenate/1 -> Orientation/1
  Matrix Concatenate1/1 -> Position/1
  Selector4/1 -> Gain/1
  Selector3/1 -> Matrix Concatenate1/1
  Pose/1 -> Selector1/1, Selector4/1, Selector3/1

== system MOBATSim/Vehicle Model 4/Vehicle Model ==
  Longitudinal Speed : Inport
  Steering Angle : Inport  Port=2
  Delay : Delay  DelayLength=1  SampleTime=Sim_Ts
  Kinematic Bicycle Model : Subsystem
  Selector3 : Selector  InputPortWidth=3  IndexOptions=Index vector (dialog)  Indices=[1]  OutputSizes=1
  Selector4 : Selector  InputPortWidth=3  IndexOptions=Index vector (dialog)  Indices=[2]  OutputSizes=1
  Sqrt : Sqrt  SaturateOnIntegerOverflow=on
  Square : Math  Operator=square  SaturateOnIntegerOverflow=on
  Square1 : Math  Operator=square  SaturateOnIntegerOverflow=on
  Sum1 : Sum  Inputs=|++
  Zero-Order Hold1 : ZeroOrderHold  SampleTime=Sim_Ts
  Zero-Order Hold2 : ZeroOrderHold  SampleTime=Sim_Ts
  Pose : Outport
  Speed : Outport  Port=2
  wires:
  Delay/1 -> Speed/1
  Kinematic Bicycle Model/1(state) -> Zero-Order Hold1/1
  Selector4/1 -> Square1/1
  Longitudinal Speed/1 -> Kinematic Bicycle Model/1(v)
  Steering Angle/1 -> Kinematic Bicycle Model/2(Steering Angle)
  Sum1/1 -> Sqrt/1
  Sqrt/1 -> Delay/1
  Square/1 -> Sum1/1
  Square1/1 -> Sum1/2
  Selector3/1 -> Square/1
  Kinematic Bicycle Model/2(stateDot) -> Zero-Order Hold2/1
  Zero-Order Hold1/1 -> Pose/1
  Zero-Order Hold2/1 -> Selector4/1, Selector3/1

== system MOBATSim/Vehicle Model 4/Vehicle Status Check and Acceleration to Speed ==
  note: Longitudinal
  Reference Acceleration : Inport
  Reference Steering Angle : Inport  Port=2
  Acceleration to Speed : Integrator  LimitOutput=on  LowerSaturationLimit=0
  MATLAB System : MATLABSystem  System=VehicleStopStatusCheck  Vehicle_id=Vehicle_id  SimulateUsing=Interpreted execution
      mask Type: VehicleStopStatusCheck
      mask Display:
      | disp('VehicleStopStatusCheck');
      | port_label('input',1,'Acc');
      | port_label('input',2,'Steering');
      | port_label('output',1,'Acc');
      | port_label('output',2,'Stop');
      | port_label('output',3,'Steering');
  Product : Product
  Signal Specification : SignalSpecification  Dimensions=1
  Stop Check : simulink/Logic and Bit Operations/Compare To Constant  relop=~=  const=1  OutDataTypeStr=uint8
  Zero-Order Hold : ZeroOrderHold  SampleTime=Sim_Ts
  Speed Cmd : Outport
  Steering Angle Cmd : Outport  Port=2
  wires:
  Acceleration to Speed/1 -> Signal Specification/1
  Stop Check/1 -> Product/2
  MATLAB System/3 -> Steering Angle Cmd/1
  Signal Specification/1 -> Zero-Order Hold/1
  Reference Acceleration/1 -> MATLAB System/1
  Zero-Order Hold/1 -> Product/1
  Product/1 -> Speed Cmd/1
  MATLAB System/1 -> Acceleration to Speed/1
  Reference Steering Angle/1 -> MATLAB System/2
  MATLAB System/2 -> Stop Check/1

== system MOBATSim/Vehicle Model 5/Longitudinal and Lateral Controllers ==
  Speed Reference : Inport
  Inter Vehicular Distance : Inport  Port=2
  Lead Speed : Inport  Port=3
  drivingMode : Inport  Port=4
  Dist2Stop : Inport  Port=5
  laneChange : Inport  Port=6
  Actual Pose : Inport  Port=7
  Actual Speed : Inport  Port=8
  Lateral Motion Control : Subsystem  Variant=on  VariantControlMode=label  LabelModeActiveChoice=STANLEY  mask{modeLateral=STANLEY}
      mask prompts: modeLateral "Lateral Control Mode:"
      mask TypeOptions modeLateral: PURE_PURSUIT | STANLEY
      mask Callback modeLateral: set_param(gcb,'OverrideUsingVariant',get_param(gcb,'modeLateral'));
  Longitudinal Speed Control : Subsystem
  Longitudinal Acceleration Cmd : Outport
  Reference Steering Angle : Outport  Port=2
  wires:
  laneChange/1 -> Lateral Motion Control/3(changeLane)
  Lateral Motion Control/1(SteerCmd) -> Reference Steering Angle/1
  Actual Speed/1 -> Lateral Motion Control/1(speed), Longitudinal Speed Control/6(Actual Speed)
  drivingMode/1 -> Longitudinal Speed Control/4(Driving Mode)
  Longitudinal Speed Control/1(Longitduinal Acceleration Command) -> Longitudinal Acceleration Cmd/1
  Dist2Stop/1 -> Longitudinal Speed Control/5(Dist2Stop)
  Inter Vehicular Distance/1 -> Longitudinal Speed Control/2(Inter Vehicular Distance)
  Lead Speed/1 -> Longitudinal Speed Control/3(Lead Speed)
  Speed Reference/1 -> Longitudinal Speed Control/1(Speed Reference)
  Actual Pose/1 -> Lateral Motion Control/2(pose)

== system MOBATSim/Vehicle Model 5/Path Planner ==
  note: 1) Add Subsystem or Model blocks as valid variant choices.
      | 2) You cannot connect blocks at this level. At simulation, connectivity is automatically
      | determined, based on the active variant and port name matching.
  CommunicationIDs : Inport
  Astar : Subsystem  VariantControl=Astar
  ShortestPathFinder : Subsystem  VariantControl=ShortestPathFinder
  waypointReached : Outport

== system MOBATSim/Vehicle Model 5/Transform to MOBATSim Coordinates ==
  Pose : Inport
  Constant : Constant  Value=0
  Constant1 : Constant
  Constant2 : Constant  Value=0
  Constant3 : Constant  Value=0
  Constant4 : Constant  Value=pi/2
  Gain : Gain  Gain=-1
  Matrix Concatenate : Concatenate  NumInputs=4  ConcatenateDimension=2
  Matrix Concatenate1 : Concatenate  NumInputs=3  ConcatenateDimension=2
  Selector1 : Selector  InputPortWidth=3  IndexOptions=Index vector (dialog)  Indices=[3]  OutputSizes=1
  Selector3 : Selector  InputPortWidth=3  IndexOptions=Index vector (dialog)  Indices=[1]  OutputSizes=1
  Selector4 : Selector  InputPortWidth=3  IndexOptions=Index vector (dialog)  Indices=[2]  OutputSizes=1
  Sum : Sum  Inputs=|++
  Position : Outport
  Orientation : Outport  Port=2
  wires:
  Sum/1 -> Matrix Concatenate/4
  Constant2/1 -> Matrix Concatenate/1
  Constant3/1 -> Matrix Concatenate1/2
  Gain/1 -> Matrix Concatenate1/3
  Constant4/1 -> Sum/2
  Constant1/1 -> Matrix Concatenate/2
  Selector1/1 -> Sum/1
  Constant/1 -> Matrix Concatenate/3
  Matrix Concatenate/1 -> Orientation/1
  Matrix Concatenate1/1 -> Position/1
  Selector4/1 -> Gain/1
  Selector3/1 -> Matrix Concatenate1/1
  Pose/1 -> Selector1/1, Selector4/1, Selector3/1

== system MOBATSim/Vehicle Model 5/Vehicle Model ==
  Longitudinal Speed : Inport
  Steering Angle : Inport  Port=2
  Delay : Delay  DelayLength=1  SampleTime=Sim_Ts
  Kinematic Bicycle Model : Subsystem
  Selector3 : Selector  InputPortWidth=3  IndexOptions=Index vector (dialog)  Indices=[1]  OutputSizes=1
  Selector4 : Selector  InputPortWidth=3  IndexOptions=Index vector (dialog)  Indices=[2]  OutputSizes=1
  Sqrt : Sqrt  SaturateOnIntegerOverflow=on
  Square : Math  Operator=square  SaturateOnIntegerOverflow=on
  Square1 : Math  Operator=square  SaturateOnIntegerOverflow=on
  Sum1 : Sum  Inputs=|++
  Zero-Order Hold1 : ZeroOrderHold  SampleTime=Sim_Ts
  Zero-Order Hold2 : ZeroOrderHold  SampleTime=Sim_Ts
  Pose : Outport
  Speed : Outport  Port=2
  wires:
  Delay/1 -> Speed/1
  Kinematic Bicycle Model/1(state) -> Zero-Order Hold1/1
  Selector4/1 -> Square1/1
  Longitudinal Speed/1 -> Kinematic Bicycle Model/1(v)
  Steering Angle/1 -> Kinematic Bicycle Model/2(Steering Angle)
  Sum1/1 -> Sqrt/1
  Sqrt/1 -> Delay/1
  Square/1 -> Sum1/1
  Square1/1 -> Sum1/2
  Selector3/1 -> Square/1
  Kinematic Bicycle Model/2(stateDot) -> Zero-Order Hold2/1
  Zero-Order Hold1/1 -> Pose/1
  Zero-Order Hold2/1 -> Selector4/1, Selector3/1

== system MOBATSim/Vehicle Model 5/Vehicle Status Check and Acceleration to Speed ==
  note: Longitudinal
  Reference Acceleration : Inport
  Reference Steering Angle : Inport  Port=2
  Acceleration to Speed : Integrator  LimitOutput=on  LowerSaturationLimit=0
  MATLAB System : MATLABSystem  System=VehicleStopStatusCheck  Vehicle_id=Vehicle_id  SimulateUsing=Interpreted execution
      mask Type: VehicleStopStatusCheck
      mask Display:
      | disp('VehicleStopStatusCheck');
      | port_label('input',1,'Acc');
      | port_label('input',2,'Steering');
      | port_label('output',1,'Acc');
      | port_label('output',2,'Stop');
      | port_label('output',3,'Steering');
  Product : Product
  Signal Specification : SignalSpecification  Dimensions=1
  Stop Check : simulink/Logic and Bit Operations/Compare To Constant  relop=~=  const=1  OutDataTypeStr=uint8
  Zero-Order Hold : ZeroOrderHold  SampleTime=Sim_Ts
  Speed Cmd : Outport
  Steering Angle Cmd : Outport  Port=2
  wires:
  Acceleration to Speed/1 -> Signal Specification/1
  Stop Check/1 -> Product/2
  MATLAB System/3 -> Steering Angle Cmd/1
  Signal Specification/1 -> Zero-Order Hold/1
  Reference Acceleration/1 -> MATLAB System/1
  Zero-Order Hold/1 -> Product/1
  Product/1 -> Speed Cmd/1
  MATLAB System/1 -> Acceleration to Speed/1
  Reference Steering Angle/1 -> MATLAB System/2
  MATLAB System/2 -> Stop Check/1

== system MOBATSim/Vehicle Model 6/Longitudinal and Lateral Controllers ==
  Speed Reference : Inport
  Inter Vehicular Distance : Inport  Port=2
  Lead Speed : Inport  Port=3
  drivingMode : Inport  Port=4
  Dist2Stop : Inport  Port=5
  laneChange : Inport  Port=6
  Actual Pose : Inport  Port=7
  Actual Speed : Inport  Port=8
  Lateral Motion Control : Subsystem  Variant=on  VariantControlMode=label  LabelModeActiveChoice=STANLEY  mask{modeLateral=STANLEY}
      mask prompts: modeLateral "Lateral Control Mode:"
      mask TypeOptions modeLateral: PURE_PURSUIT | STANLEY
      mask Callback modeLateral: set_param(gcb,'OverrideUsingVariant',get_param(gcb,'modeLateral'));
  Longitudinal Speed Control : Subsystem
  Longitudinal Acceleration Cmd : Outport
  Reference Steering Angle : Outport  Port=2
  wires:
  laneChange/1 -> Lateral Motion Control/3(changeLane)
  Lateral Motion Control/1(SteerCmd) -> Reference Steering Angle/1
  Actual Speed/1 -> Lateral Motion Control/1(speed), Longitudinal Speed Control/6(Actual Speed)
  drivingMode/1 -> Longitudinal Speed Control/4(Driving Mode)
  Longitudinal Speed Control/1(Longitduinal Acceleration Command) -> Longitudinal Acceleration Cmd/1
  Dist2Stop/1 -> Longitudinal Speed Control/5(Dist2Stop)
  Inter Vehicular Distance/1 -> Longitudinal Speed Control/2(Inter Vehicular Distance)
  Lead Speed/1 -> Longitudinal Speed Control/3(Lead Speed)
  Speed Reference/1 -> Longitudinal Speed Control/1(Speed Reference)
  Actual Pose/1 -> Lateral Motion Control/2(pose)

== system MOBATSim/Vehicle Model 6/Path Planner ==
  note: 1) Add Subsystem or Model blocks as valid variant choices.
      | 2) You cannot connect blocks at this level. At simulation, connectivity is automatically
      | determined, based on the active variant and port name matching.
  CommunicationIDs : Inport
  Astar : Subsystem  VariantControl=Astar
  ShortestPathFinder : Subsystem  VariantControl=ShortestPathFinder
  waypointReached : Outport

== system MOBATSim/Vehicle Model 6/Transform to MOBATSim Coordinates ==
  Pose : Inport
  Constant : Constant  Value=0
  Constant1 : Constant
  Constant2 : Constant  Value=0
  Constant3 : Constant  Value=0
  Constant4 : Constant  Value=pi/2
  Gain : Gain  Gain=-1
  Matrix Concatenate : Concatenate  NumInputs=4  ConcatenateDimension=2
  Matrix Concatenate1 : Concatenate  NumInputs=3  ConcatenateDimension=2
  Selector1 : Selector  InputPortWidth=3  IndexOptions=Index vector (dialog)  Indices=[3]  OutputSizes=1
  Selector3 : Selector  InputPortWidth=3  IndexOptions=Index vector (dialog)  Indices=[1]  OutputSizes=1
  Selector4 : Selector  InputPortWidth=3  IndexOptions=Index vector (dialog)  Indices=[2]  OutputSizes=1
  Sum : Sum  Inputs=|++
  Position : Outport
  Orientation : Outport  Port=2
  wires:
  Sum/1 -> Matrix Concatenate/4
  Constant2/1 -> Matrix Concatenate/1
  Constant3/1 -> Matrix Concatenate1/2
  Gain/1 -> Matrix Concatenate1/3
  Constant4/1 -> Sum/2
  Constant1/1 -> Matrix Concatenate/2
  Selector1/1 -> Sum/1
  Constant/1 -> Matrix Concatenate/3
  Matrix Concatenate/1 -> Orientation/1
  Matrix Concatenate1/1 -> Position/1
  Selector4/1 -> Gain/1
  Selector3/1 -> Matrix Concatenate1/1
  Pose/1 -> Selector1/1, Selector4/1, Selector3/1

== system MOBATSim/Vehicle Model 6/Vehicle Model ==
  Longitudinal Speed : Inport
  Steering Angle : Inport  Port=2
  Delay : Delay  DelayLength=1  SampleTime=Sim_Ts
  Kinematic Bicycle Model : Subsystem
  Selector3 : Selector  InputPortWidth=3  IndexOptions=Index vector (dialog)  Indices=[1]  OutputSizes=1
  Selector4 : Selector  InputPortWidth=3  IndexOptions=Index vector (dialog)  Indices=[2]  OutputSizes=1
  Sqrt : Sqrt  SaturateOnIntegerOverflow=on
  Square : Math  Operator=square  SaturateOnIntegerOverflow=on
  Square1 : Math  Operator=square  SaturateOnIntegerOverflow=on
  Sum1 : Sum  Inputs=|++
  Zero-Order Hold1 : ZeroOrderHold  SampleTime=Sim_Ts
  Zero-Order Hold2 : ZeroOrderHold  SampleTime=Sim_Ts
  Pose : Outport
  Speed : Outport  Port=2
  wires:
  Delay/1 -> Speed/1
  Kinematic Bicycle Model/1(state) -> Zero-Order Hold1/1
  Selector4/1 -> Square1/1
  Longitudinal Speed/1 -> Kinematic Bicycle Model/1(v)
  Steering Angle/1 -> Kinematic Bicycle Model/2(Steering Angle)
  Sum1/1 -> Sqrt/1
  Sqrt/1 -> Delay/1
  Square/1 -> Sum1/1
  Square1/1 -> Sum1/2
  Selector3/1 -> Square/1
  Kinematic Bicycle Model/2(stateDot) -> Zero-Order Hold2/1
  Zero-Order Hold1/1 -> Pose/1
  Zero-Order Hold2/1 -> Selector4/1, Selector3/1

== system MOBATSim/Vehicle Model 6/Vehicle Status Check and Acceleration to Speed ==
  note: Longitudinal
  Reference Acceleration : Inport
  Reference Steering Angle : Inport  Port=2
  Acceleration to Speed : Integrator  LimitOutput=on  LowerSaturationLimit=0
  MATLAB System : MATLABSystem  System=VehicleStopStatusCheck  Vehicle_id=Vehicle_id  SimulateUsing=Interpreted execution
      mask Type: VehicleStopStatusCheck
      mask Display:
      | disp('VehicleStopStatusCheck');
      | port_label('input',1,'Acc');
      | port_label('input',2,'Steering');
      | port_label('output',1,'Acc');
      | port_label('output',2,'Stop');
      | port_label('output',3,'Steering');
  Product : Product
  Signal Specification : SignalSpecification  Dimensions=1
  Stop Check : simulink/Logic and Bit Operations/Compare To Constant  relop=~=  const=1  OutDataTypeStr=uint8
  Zero-Order Hold : ZeroOrderHold  SampleTime=Sim_Ts
  Speed Cmd : Outport
  Steering Angle Cmd : Outport  Port=2
  wires:
  Acceleration to Speed/1 -> Signal Specification/1
  Stop Check/1 -> Product/2
  MATLAB System/3 -> Steering Angle Cmd/1
  Signal Specification/1 -> Zero-Order Hold/1
  Reference Acceleration/1 -> MATLAB System/1
  Zero-Order Hold/1 -> Product/1
  Product/1 -> Speed Cmd/1
  MATLAB System/1 -> Acceleration to Speed/1
  Reference Steering Angle/1 -> MATLAB System/2
  MATLAB System/2 -> Stop Check/1

== system MOBATSim/Vehicle Model 7/Longitudinal and Lateral Controllers ==
  Speed Reference : Inport
  Inter Vehicular Distance : Inport  Port=2
  Lead Speed : Inport  Port=3
  drivingMode : Inport  Port=4
  Dist2Stop : Inport  Port=5
  laneChange : Inport  Port=6
  Actual Pose : Inport  Port=7
  Actual Speed : Inport  Port=8
  Lateral Motion Control : Subsystem  Variant=on  VariantControlMode=label  LabelModeActiveChoice=STANLEY  mask{modeLateral=STANLEY}
      mask prompts: modeLateral "Lateral Control Mode:"
      mask TypeOptions modeLateral: PURE_PURSUIT | STANLEY
      mask Callback modeLateral: set_param(gcb,'OverrideUsingVariant',get_param(gcb,'modeLateral'));
  Longitudinal Speed Control : Subsystem
  Longitudinal Acceleration Cmd : Outport
  Reference Steering Angle : Outport  Port=2
  wires:
  laneChange/1 -> Lateral Motion Control/3(changeLane)
  Lateral Motion Control/1(SteerCmd) -> Reference Steering Angle/1
  Actual Speed/1 -> Lateral Motion Control/1(speed), Longitudinal Speed Control/6(Actual Speed)
  drivingMode/1 -> Longitudinal Speed Control/4(Driving Mode)
  Longitudinal Speed Control/1(Longitduinal Acceleration Command) -> Longitudinal Acceleration Cmd/1
  Dist2Stop/1 -> Longitudinal Speed Control/5(Dist2Stop)
  Inter Vehicular Distance/1 -> Longitudinal Speed Control/2(Inter Vehicular Distance)
  Lead Speed/1 -> Longitudinal Speed Control/3(Lead Speed)
  Speed Reference/1 -> Longitudinal Speed Control/1(Speed Reference)
  Actual Pose/1 -> Lateral Motion Control/2(pose)

== system MOBATSim/Vehicle Model 7/Path Planner ==
  note: 1) Add Subsystem or Model blocks as valid variant choices.
      | 2) You cannot connect blocks at this level. At simulation, connectivity is automatically
      | determined, based on the active variant and port name matching.
  CommunicationIDs : Inport
  Astar : Subsystem  VariantControl=Astar
  ShortestPathFinder : Subsystem  VariantControl=ShortestPathFinder
  waypointReached : Outport

== system MOBATSim/Vehicle Model 7/Transform to MOBATSim Coordinates ==
  Pose : Inport
  Constant : Constant  Value=0
  Constant1 : Constant
  Constant2 : Constant  Value=0
  Constant3 : Constant  Value=0
  Constant4 : Constant  Value=pi/2
  Gain : Gain  Gain=-1
  Matrix Concatenate : Concatenate  NumInputs=4  ConcatenateDimension=2
  Matrix Concatenate1 : Concatenate  NumInputs=3  ConcatenateDimension=2
  Selector1 : Selector  InputPortWidth=3  IndexOptions=Index vector (dialog)  Indices=[3]  OutputSizes=1
  Selector3 : Selector  InputPortWidth=3  IndexOptions=Index vector (dialog)  Indices=[1]  OutputSizes=1
  Selector4 : Selector  InputPortWidth=3  IndexOptions=Index vector (dialog)  Indices=[2]  OutputSizes=1
  Sum : Sum  Inputs=|++
  Position : Outport
  Orientation : Outport  Port=2
  wires:
  Sum/1 -> Matrix Concatenate/4
  Constant2/1 -> Matrix Concatenate/1
  Constant3/1 -> Matrix Concatenate1/2
  Gain/1 -> Matrix Concatenate1/3
  Constant4/1 -> Sum/2
  Constant1/1 -> Matrix Concatenate/2
  Selector1/1 -> Sum/1
  Constant/1 -> Matrix Concatenate/3
  Matrix Concatenate/1 -> Orientation/1
  Matrix Concatenate1/1 -> Position/1
  Selector4/1 -> Gain/1
  Selector3/1 -> Matrix Concatenate1/1
  Pose/1 -> Selector1/1, Selector4/1, Selector3/1
